simulink model "FullFMS_2026_02_25_V0_4_25_R2025b"  (R2025b)
settings: Solver=FixedStepAuto  StopTime=inf  FixedStep=0.01  MaxStep=0.01  RelTol=1e-2
PreLoadFcn:
  | load("BUS_CONFIG.mat")
libraries: opcualib x8
(part 2 of 4)

== matlab function FullFMS_2026_02_25_V0_4_25_R2025b/MATLAB Function6 ==
  data: F_92_Claw_2_Cart output boolean; F_92_Claw_2_Del output boolean; F_92_Claw_Down output boolean; F_92_Close_Claw output boolean; F_93_Led_Start output boolean; F_93_Led_Reset output boolean; F_93_Led_Extra1 output boolean; F_93_Led_Extra2 output boolean; F_93_Panel_O4 output boolean; F_93_Panel_O5 output boolean; F_93_Panel_O6 output boolean; F_93_Panel_O7 output boolean; u1 input boolean; A_94_Request output boolean; u2 input boolean; u3 input boolean; u4 input boolean; u5 input boolean; u6 input boolean; u7 input boolean; u8 input boolean; u9 input boolean; u10 input boolean; u11 input boolean; u12 input boolean; u13 input boolean; u14 input boolean; u15 input boolean; u16 input boolean; u17 input double; u18 input boolean; u19 input boolean; u20 input boolean; u21 input boolean; u22 input boolean; u23 input boolean; u24 input boolean; u25 input boolean; u26 input boolean; u27 input boolean; u28 input boolean; u29 input boolean; u30 input boolean; u31 input boolean; u32 input boolean; u33 input boolean; u34 input boolean; u35 input boolean; u36 input boolean; u37 input boolean; u38 input boolean; u39 input boolean; u40 input boolean; u41 input boolean; u42 input boolean; u43 input boolean; u44 input boolean; u45 input boolean; u46 input boolean; A_94_No_Cart output boolean; A_94_Cart_Full output boolean; A_94_CRoute_Out output boolean; A_93_ProcCartID output double; A_94_Cart_Stat output boolean; A_94_Cart_Next output boolean; A_94_Optic output boolean; A_94_Count output boolean; A_94_Pist_Bck output boolean; A_94_Release_FB output boolean; A_94_CRoute_In output boolean; C_95_Initialization output boolean; C_95_PD_Proc output boolean; C_95_PD_Cart output boolean; C_92_Profibus output boolean; C_95_Start output boolean; C_95_Cart2Del output boolean; C_95_Del2Cart output boolean; O_90_Part_Reserve output boolean; O_90_Claw_Del output boolean; O_90_Claw_Cart output boolean; O_90_Claw_Reserve output boolean; O_90_Claw_Low output boolean; O_90_Claw_High output boolean; O_90_Part_in_Claw output boolean; O_91_Start output boolean; O_91_Stop output boolean; O_91_Key_Pos output boolean; O_91_Reset output boolean; O_91_Panel_I4 output boolean; O_91_Panel_I5 output boolean; O_91_Panel_I6 output boolean; O_91_Panel_I7 output boolean
function [F_92_Claw_2_Cart,F_92_Claw_2_Del,F_92_Claw_Down,F_92_Close_Claw,F_93_Led_Start,F_93_Led_Reset,F_93_Led_Extra1,F_93_Led_Extra2,F_93_Panel_O4,F_93_Panel_O5,F_93_Panel_O6,F_93_Panel_O7, ...
    A_94_Request,A_94_No_Cart,A_94_Cart_Full,A_94_CRoute_Out,A_93_ProcCartID,A_94_Cart_Stat,A_94_Cart_Next,A_94_Optic,A_94_Count,A_94_Pist_Bck,A_94_Release_FB,A_94_CRoute_In, ...
    C_95_Initialization,C_95_PD_Proc,C_95_PD_Cart,C_92_Profibus,C_95_Start,C_95_Cart2Del,C_95_Del2Cart, ...
    O_90_Part_Reserve,O_90_Claw_Del,O_90_Claw_Cart,O_90_Claw_Reserve,O_90_Claw_Low,O_90_Claw_High,O_90_Part_in_Claw,O_91_Start,O_91_Stop,O_91_Key_Pos,O_91_Reset,O_91_Panel_I4,O_91_Panel_I5,O_91_Panel_I6,O_91_Panel_I7] = ...
    Handling2_90(u1, u2, u3, u4, u5, u6, u7, u8, u9, u10, u11, u12, u13, u14, u15, u16, u17, u18, u19, u20, u21, u22, u23, u24, u25, u26, u27, u28, u29, u30, u31, u32, u33, u34, u35, u36, u37, u38, u39, u40, u41, u42, u43, u44, u45, u46)

% Actuators (12 variables, starts at u1)
F_92_Claw_2_Cart = u1;
F_92_Claw_2_Del = u2;
F_92_Claw_Down = u3;
F_92_Close_Claw = u4;
F_93_Led_Start = u5;
F_93_Led_Reset = u6;
F_93_Led_Extra1 = u7;
F_93_Led_Extra2 = u8;
F_93_Panel_O4 = u9;
F_93_Panel_O5 = u10;
F_93_Panel_O6 = u11;
F_93_Panel_O7 = u12;

% AS-i (12 variables, starts at u13)
A_94_Request = u13;
A_94_No_Cart = u14;
A_94_Cart_Full = u15;
A_94_CRoute_Out = u16;
A_93_ProcCartID = u17;
A_94_Cart_Stat = u18;
A_94_Cart_Next = u19;
A_94_Optic = u20;
A_94_Count = u21;
A_94_Pist_Bck = u22;
A_94_Release_FB = u23;
A_94_CRoute_In = u24;

% Control (7 variables, starts at u25)
C_95_Initialization = u25;
C_95_PD_Proc = u26;
C_95_PD_Cart = u27;
C_92_Profibus = u28;
C_95_Start = u29;
C_95_Cart2Del = u30;
C_95_Del2Cart = u31;

% Sensors (15 variables, starts at u32)
O_90_Part_Reserve = u32;
O_90_Claw_Del = u33;
O_90_Claw_Cart = u34;
O_90_Claw_Reserve = u35;
O_90_Claw_Low = u36;
O_90_Claw_High = u37;
O_90_Part_in_Claw = u38;
O_91_Start = u39;
O_91_Stop = u40;
O_91_Key_Pos = u41;
O_91_Reset = u42;
O_91_Panel_I4 = u43;
O_91_Panel_I5 = u44;
O_91_Panel_I6 = u45;
O_91_Panel_I7 = u46;

end

== matlab function FullFMS_2026_02_25_V0_4_25_R2025b/MATLAB Function5 ==
  data: u1 input boolean; u2 input boolean; u3 input boolean; u4 input boolean; u5 input boolean; u6 input boolean; u7 input boolean; u8 input boolean; u9 input boolean; u10 input boolean; u11 input boolean; u12 input boolean; u13 input boolean; u14 input boolean; u15 input boolean; u16 input boolean; u17 input double; u18 input double; u19 input boolean; u20 input double; u21 input boolean; u22 input boolean; u23 input boolean; u24 input boolean; u25 input boolean; u26 input boolean; u27 input boolean; u28 input boolean; u29 input boolean; u30 input boolean; u31 input boolean; u32 input boolean; u33 input boolean; u34 input boolean; u35 input boolean; u36 input boolean; u37 input boolean; u38 input boolean; u39 input boolean; F_82_Pist_Adv output boolean; F_82_Suction_On output boolean; F_82_Suction_Off output boolean; F_82_Arm_2_Del output boolean; F_82_Arm_2_Mag output boolean; F_83_Led_Start output boolean; F_83_Led_Reset output boolean; F_83_Led_Extra1 output boolean; F_83_Led_Extra2 output boolean; F_83_Panel_O4 output boolean; F_83_Panel_O5 output boolean; F_83_Panel_O6 output boolean; F_83_Panel_O7 output boolean; C_85_Initialization output boolean; C_85_Part_Del output boolean; C_85_Part_Mag output boolean; C_86_Mag_Parts output double; C_87_RQ_MParts output double; C_82_Profibus output boolean; C_83_RQ_Parts output double; C_85_Start output boolean; C_85_Single output boolean; C_85_Continuous output boolean; C_85_Counted output boolean; O_80_Mag_Full output boolean; O_80_Pist_Bck output boolean; O_80_Pist_Fwd output boolean; O_80_Part_Stuck output boolean; O_80_Arm_Mag output boolean; O_80_Arm_Del output boolean; O_80_Mag_Empty output boolean; O_81_Start output boolean; O_81_Stop output boolean; O_81_Key_Pos output boolean; O_81_Reset output boolean; O_81_Panel_I4 output boolean; O_81_Panel_I5 output boolean; O_81_Panel_I6 output boolean; O_81_Panel_I7 output boolean
function [F_82_Pist_Adv, F_82_Suction_On,F_82_Suction_Off,F_82_Arm_2_Del,F_82_Arm_2_Mag,F_83_Led_Start , F_83_Led_Reset , F_83_Led_Extra1 , F_83_Led_Extra2 , F_83_Panel_O4 , F_83_Panel_O5 , F_83_Panel_O6 , F_83_Panel_O7, ...
    C_85_Initialization,C_85_Part_Del,C_85_Part_Mag,C_86_Mag_Parts,C_87_RQ_MParts,C_82_Profibus,C_83_RQ_Parts,C_85_Start,C_85_Single,C_85_Continuous,C_85_Counted, ...
    O_80_Mag_Full,O_80_Pist_Bck,O_80_Pist_Fwd,O_80_Part_Stuck,O_80_Arm_Mag,O_80_Arm_Del,O_80_Mag_Empty,O_81_Start,O_81_Stop,O_81_Key_Pos,O_81_Reset,O_81_Panel_I4,O_81_Panel_I5,O_81_Panel_I6,O_81_Panel_I7] = ...
    Distribution_80 (u1, u2, u3, u4, u5, u6, u7, u8, u9, u10, u11, u12, u13, u14, u15, u16, u17, u18, u19, u20, u21, u22, u23, u24, u25, u26, u27, u28, u29, u30, u31, u32, u33, u34, u35, u36, u37, u38, u39)

% Actuatorss (13 variables, starts at u1)
F_82_Pist_Adv = u1;
F_82_Suction_On = u2;
F_82_Suction_Off = u3;
F_82_Arm_2_Del = u4;
F_82_Arm_2_Mag = u5;
F_83_Led_Start = u6;
F_83_Led_Reset = u7;
F_83_Led_Extra1 = u8;
F_83_Led_Extra2 = u9;
F_83_Panel_O4 = u10;
F_83_Panel_O5 = u11;
F_83_Panel_O6 = u12;
F_83_Panel_O7 = u13;

% Control (11 varaibles, starts at u14)
C_85_Initialization = u14;
C_85_Part_Del = u15;
C_85_Part_Mag = u16;
C_86_Mag_Parts = u17;
C_87_RQ_MParts = u18;
C_82_Profibus = u19;
C_83_RQ_Parts = u20;
C_85_Start = u21;
C_85_Single = u22;
C_85_Continuous = u23;
C_85_Counted = u24;

% Sensors (15 variables, starts at u25)
O_80_Mag_Full = u25;
O_80_Pist_Bck = u26;
O_80_Pist_Fwd = u27;
O_80_Part_Stuck = u28;
O_80_Arm_Mag = u29;
O_80_Arm_Del = u30;
O_80_Mag_Empty = u31;
O_81_Start = u32;
O_81_Stop = u33;
O_81_Key_Pos = u34;
O_81_Reset = u35;
O_81_Panel_I4 = u36;
O_81_Panel_I5 = u37;
O_81_Panel_I6 = u38;
O_81_Panel_I7 = u39;

end

== matlab function FullFMS_2026_02_25_V0_4_25_R2025b/MATLAB Function4 ==
  data: u1 input boolean; u2 input boolean; u3 input boolean; u4 input boolean; u5 input boolean; u6 input boolean; u7 input boolean; u8 input boolean; u9 input boolean; u10 input boolean; u11 input boolean; u12 input boolean; u13 input boolean; u14 input boolean; u15 input boolean; u16 input boolean; u17 input boolean; u18 input double; u19 input boolean; u20 input boolean; u21 input boolean; u22 input boolean; u23 input boolean; u24 input boolean; u25 input boolean; u26 input boolean; u27 input boolean; u28 input boolean; u29 input boolean; u30 input boolean; u31 input boolean; u32 input boolean; u33 input boolean; u34 input boolean; u35 input boolean; u36 input boolean; u37 input boolean; u38 input boolean; u39 input boolean; u40 input boolean; u41 input boolean; u42 input boolean; u43 input boolean; u44 input boolean; u45 input boolean; u46 input boolean; u47 input boolean; u48 input boolean; u49 input boolean; u50 input boolean; u51 input boolean; u52 input boolean; u53 input boolean; F_72_Elev_Down output boolean; F_72_Elev_Up output boolean; F_72_Eject_Part output boolean; F_72_Air_On output boolean; F_73_Led_Start output boolean; F_73_Led_Reset output boolean; F_73_Led_Extra1 output boolean; F_73_Led_Extra2 output boolean; F_73_Panel_O4 output boolean; F_73_Panel_O5 output boolean; F_73_Panel_O6 output boolean; F_73_Panel_O7 output boolean; A_74_Request output boolean; A_74_No_Cart output boolean; A_74_Cart_Full output boolean; A_74_CRoute_Out output boolean; A_74_CRoute_In80 output boolean; A_73_TestCartID output double; A_74_Cart_Stat output boolean; A_74_Cart_Next output boolean; A_74_Optic output boolean; A_74_Count output boolean; A_74_Pist_Bck output boolean; A_74_Release_FB output boolean; A_74_CRoute_In output boolean; C_75_Initialization output boolean; C_75_ID_Delivery1 output boolean; C_75_ID_Delivery2 output boolean; C_75_Part_Del output boolean; C_75_RQ_Part_Del output boolean; C_75_RQ_Wrong output boolean; C_75_Identified80 output boolean; C_75_Requested80 output boolean; C_72_Profibus output boolean; C_75_RQ_Delivery1 output boolean; C_75_RQ_Delivery2 output boolean; C_75_Identified output boolean; C_75_Requested output boolean; O_70_SInductive output boolean; O_70_SPart output boolean; O_70_SStation output boolean; O_70_SPart_Height output boolean; O_70_Elev_High output boolean; O_70_Elev_Low output boolean; O_70_Pist_Bck output boolean; O_71_Start output boolean; O_71_Stop output boolean; O_71_Key_Pos output boolean; O_71_Reset output boolean; O_71_Panel_I4 output boolean; O_71_Panel_I5 output boolean; O_71_Panel_I6 output boolean; O_71_Panel_I7 output boolean
function [F_72_Elev_Down,F_72_Elev_Up,F_72_Eject_Part,F_72_Air_On,F_73_Led_Start,F_73_Led_Reset,F_73_Led_Extra1,F_73_Led_Extra2,F_73_Panel_O4,F_73_Panel_O5,F_73_Panel_O6,F_73_Panel_O7, ...	
    A_74_Request,A_74_No_Cart,A_74_Cart_Full,A_74_CRoute_Out,A_74_CRoute_In80,A_73_TestCartID,A_74_Cart_Stat,A_74_Cart_Next,A_74_Optic,A_74_Count,A_74_Pist_Bck,A_74_Release_FB,A_74_CRoute_In, ...
    C_75_Initialization,C_75_ID_Delivery1,C_75_ID_Delivery2,C_75_Part_Del,C_75_RQ_Part_Del,C_75_RQ_Wrong,C_75_Identified80,C_75_Requested80,C_72_Profibus,C_75_RQ_Delivery1,C_75_RQ_Delivery2,C_75_Identified , C_75_Requested, ...
    O_70_SInductive,O_70_SPart,O_70_SStation,O_70_SPart_Height,O_70_Elev_High,O_70_Elev_Low,O_70_Pist_Bck,O_71_Start,O_71_Stop,O_71_Key_Pos,O_71_Reset,O_71_Panel_I4,O_71_Panel_I5,O_71_Panel_I6,O_71_Panel_I7] = ...
    Testing_70(u1, u2, u3, u4, u5, u6, u7, u8, u9, u10, u11, u12, u13, u14, u15, u16, u17, u18, u19, u20, u21, u22, u23, u24, u25, u26, u27, u28, u29, u30, u31, u32, u33, u34, u35, u36, u37, u38, u39, u40, u41, u42, u43, u44, u45, u46, u47, u48, u49, u50, u51, u52, u53)

% Actuators (12 variables, starts at u1)
F_72_Elev_Down = u1;
F_72_Elev_Up = u2;
F_72_Eject_Part = u3;
F_72_Air_On = u4;
F_73_Led_Start = u5;
F_73_Led_Reset = u6;
F_73_Led_Extra1 = u7;
F_73_Led_Extra2 = u8;
F_73_Panel_O4 = u9;
F_73_Panel_O5 = u10;
F_73_Panel_O6 = u11;
F_73_Panel_O7 = u12;

% AS-i (13 varaibles, starts at u13)
A_74_Request = u13;
A_74_No_Cart = u14;
A_74_Cart_Full = u15;
A_74_CRoute_Out = u16;
A_74_CRoute_In80 = u17;
A_73_TestCartID = u18;
A_74_Cart_Stat = u19;
A_74_Cart_Next = u20;
A_74_Optic = u21;
A_74_Count = u22;
A_74_Pist_Bck = u23;
A_74_Release_FB = u24;
A_74_CRoute_In = u25;

% Control (13 variables, starts at u26)
C_75_Initialization = u26;
C_75_ID_Delivery1 = u27;
C_75_ID_Delivery2 = u28;
C_75_Part_Del = u29;
C_75_RQ_Part_Del = u30;
C_75_RQ_Wrong = u31;
C_75_Identified80 = u32;
C_75_Requested80 = u33;
C_72_Profibus = u34;
C_75_RQ_Delivery1 = u35;
C_75_RQ_Delivery2 = u36;
C_75_Identified = u37;
C_75_Requested = u38;

% Sensors (15 variables, starts at u39)
O_70_SInductive = u39;
O_70_SPart = u40;
O_70_SStation = u41;
O_70_SPart_Height = u42;
O_70_Elev_High = u43;
O_70_Elev_Low = u44;
O_70_Pist_Bck = u45;
O_71_Start = u46;
O_71_Stop = u47;
O_71_Key_Pos = u48;
O_71_Reset = u49;
O_71_Panel_I4 = u50;
O_71_Panel_I5 = u51;
O_71_Panel_I6 = u52;
O_71_Panel_I7 = u53;

end

== matlab function FullFMS_2026_02_25_V0_4_25_R2025b/MATLAB Function7 ==
  data: F_102_Drill_On output boolean; F_102_RT_On output boolean; F_102_Drill_Down output boolean; F_102_Drill_Up output boolean; F_102_Drill_Pin output boolean; F_102_Test_Pin output boolean; F_103_Led_Start output boolean; F_103_Led_Reset output boolean; F_103_Led_Extra1 output boolean; F_103_Led_Extra2 output boolean; F_103_Panel_O4 output boolean; F_103_Panel_O5 output boolean; F_103_Panel_O6 output boolean; F_103_Panel_O7 output boolean; u1 input boolean; C_105_Initialization output boolean; u2 input boolean; u3 input boolean; u4 input boolean; u5 input boolean; u6 input boolean; u7 input boolean; u8 input boolean; u9 input boolean; u10 input boolean; u11 input boolean; u12 input boolean; u13 input boolean; u14 input boolean; u15 input boolean; u16 input boolean; u17 input boolean; u18 input boolean; u19 input double; u20 input boolean; u21 input double; u22 input boolean; u23 input boolean; u24 input boolean; u25 input boolean; u26 input boolean; u27 input boolean; u28 input boolean; u29 input boolean; u30 input boolean; u31 input boolean; u32 input boolean; u33 input boolean; u34 input boolean; u35 input boolean; u36 input boolean; u37 input boolean; u38 input boolean; u39 input boolean; C_105_Part_ready output boolean; C_105_Test_Ok output boolean; C_105_Test_Fail output boolean; C_106_RT_Counter output double; C_102_Profibus output boolean; C_103_RQ_Turns output double; C_105_Start output boolean; C_105_Test output boolean; C_105_TestDrill output boolean; C_105_Rotation output boolean; O_100_PInit_Pos output boolean; O_100_PDrill_Pos output boolean; O_100_PTest_Pos output boolean; O_100_SDrill_High output boolean; O_100_SDrill_Low output boolean; O_100_RT_Sensor output boolean; O_100_PTest_Ok output boolean; O_101_Start output boolean; O_101_Stop output boolean; O_101_Key_Pos output boolean; O_101_Reset output boolean; O_101_Panel_I4 output boolean; O_101_Panel_I5 output boolean; O_101_Panel_I6 output boolean; O_101_Panel_I7 output boolean; u40 input boolean
function [F_102_Drill_On,F_102_RT_On,F_102_Drill_Down,F_102_Drill_Up,F_102_Drill_Pin,F_102_Test_Pin,F_103_Led_Start,F_103_Led_Reset,F_103_Led_Extra1,F_103_Led_Extra2,F_103_Panel_O4,F_103_Panel_O5,F_103_Panel_O6,F_103_Panel_O7, ...
    C_105_Initialization,C_105_Part_ready,C_105_Test_Ok,C_105_Test_Fail,C_106_RT_Counter,C_102_Profibus,C_103_RQ_Turns,C_105_Start,C_105_Test,C_105_TestDrill,C_105_Rotation, ...
    O_100_PInit_Pos,O_100_PDrill_Pos,O_100_PTest_Pos,O_100_SDrill_High,O_100_SDrill_Low,O_100_RT_Sensor,O_100_PTest_Ok,O_101_Start,O_101_Stop,O_101_Key_Pos,O_101_Reset,O_101_Panel_I4,O_101_Panel_I5,O_101_Panel_I6,O_101_Panel_I7] = ...
    Processing_100(u1, u2, u3, u4, u5, u6, u7, u8, u9, u10, u11, u12, u13, u14, u15, u16, u17, u18, u19, u20, u21, u22, u23, u24, u25, u26, u27, u28, u29, u30, u31, u32, u33, u34, u35, u36, u37, u38, u39, u40)

% Actuators (14 variables, starts at u1)
F_102_Drill_On = u1;
F_102_RT_On = u2;
F_102_Drill_Down = u3;
F_102_Drill_Up = u4;
F_102_Drill_Pin = u5;
F_102_Test_Pin = u6;
F_103_Led_Start = u7;
F_103_Led_Reset = u8;
F_103_Led_Extra1 = u9;
F_103_Led_Extra2 = u10;
F_103_Panel_O4 = u11;
F_103_Panel_O5 = u12;
F_103_Panel_O6 = u13;
F_103_Panel_O7 = u14;

% Control (11 variables, starting at u15)
C_105_Initialization = u15;
C_105_Part_ready = u16;
C_105_Test_Ok = u17;
C_105_Test_Fail = u18;
C_106_RT_Counter = u19;
C_102_Profibus = u20;
C_103_RQ_Turns = u21;
C_105_Start = u22;
C_105_Test = u23;
C_105_TestDrill = u24;
C_105_Rotation = u25;

% Sensors (15 variables, starts at u26)
O_100_PInit_Pos = u26;
O_100_PDrill_Pos = u27;
O_100_PTest_Pos = u28;
O_100_SDrill_High = u29;
O_100_SDrill_Low = u30;
O_100_RT_Sensor = u31;
O_100_PTest_Ok = u32;
O_101_Start = u33;
O_101_Stop = u34;
O_101_Key_Pos = u35;
O_101_Reset = u36;
O_101_Panel_I4 = u37;
O_101_Panel_I5 = u38;
O_101_Panel_I6 = u39;
O_101_Panel_I7 = u40;

end

== matlab function FullFMS_2026_02_25_V0_4_25_R2025b/MATLAB Function8 ==
  data: u1 input boolean; u2 input boolean; u3 input boolean; u4 input boolean; u5 input boolean; u6 input boolean; u7 input boolean; u8 input boolean; u9 input boolean; u10 input boolean; u11 input boolean; u12 input boolean; u13 input double; u14 input boolean; u15 input boolean; u16 input boolean; u17 input boolean; u18 input boolean; u19 input boolean; u20 input boolean; u21 input boolean; u22 input boolean; u23 input boolean; u24 input boolean; u25 input boolean; u26 input boolean; u27 input boolean; u28 input boolean; u29 input boolean; u30 input boolean; u31 input boolean; u32 input boolean; u33 input boolean; F_43_Led_Start output boolean; F_43_Led_Reset output boolean; F_43_Led_Extra1 output boolean; F_43_Led_Extra2 output boolean; F_43_Panel_O4 output boolean; F_43_Panel_O5 output boolean; F_43_Panel_O6 output boolean; F_43_Panel_O7 output boolean; A_44_Request output boolean; A_44_No_Cart output boolean; A_44_Cart_Full output boolean; A_44_CRoute_Out output boolean; A_43_StorCartID output double; A_44_Cart_Stat output boolean; A_44_Cart_Next output boolean; A_44_Optic output boolean; A_44_Count output boolean; A_44_Pist_Bck output boolean; A_44_Release_FB output boolean; A_44_CRoute_In output boolean; C_45_Initialization output boolean; C_42_Profibus output boolean; C_45_Start output boolean; C_45_StorePart output boolean; C_45_RetrievePart output boolean; O_41_Start output boolean; O_41_Stop output boolean; O_41_Key_Pos output boolean; O_41_Reset output boolean; O_41_Panel_I4 output boolean; O_41_Panel_I5 output boolean; O_41_Panel_I6 output boolean; O_41_Panel_I7 output boolean
function [F_43_Led_Start,F_43_Led_Reset,F_43_Led_Extra1,F_43_Led_Extra2,F_43_Panel_O4,F_43_Panel_O5,F_43_Panel_O6,F_43_Panel_O7,...
 A_44_Request,A_44_No_Cart,A_44_Cart_Full,A_44_CRoute_Out,A_43_StorCartID,A_44_Cart_Stat,A_44_Cart_Next,A_44_Optic,A_44_Count,A_44_Pist_Bck,A_44_Release_FB,A_44_CRoute_In,...
 C_45_Initialization,C_42_Profibus,C_45_Start,C_45_StorePart,C_45_RetrievePart,...
    O_41_Start,O_41_Stop,O_41_Key_Pos,O_41_Reset,O_41_Panel_I4,O_41_Panel_I5,O_41_Panel_I6,O_41_Panel_I7] = ...
    Storage_40 (u1, u2, u3, u4, u5, u6, u7, u8, u9, u10, u11, u12, u13, u14, u15, u16, u17, u18, u19, u20, u21, u22, u23, u24, u25, u26, u27, u28, u29, u30, u31, u32, u33)

% Actuators (8 variables: starts at u1)
F_43_Led_Start = u1;
F_43_Led_Reset = u2;
F_43_Led_Extra1 = u3; 
F_43_Led_Extra2 = u4;
F_43_Panel_O4 = u5;
F_43_Panel_O5 = u6;
F_43_Panel_O6 = u7;
F_43_Panel_O7 = u8;

% AS-i (12 variables: starts at u9)
A_44_Request = u9;
A_44_No_Cart = u10;
A_44_Cart_Full = u11;
A_44_CRoute_Out = u12;
A_43_StorCartID = u13;
A_44_Cart_Stat = u14;
A_44_Cart_Next = u15;
A_44_Optic = u16;
A_44_Count = u17;
A_44_Pist_Bck = u18;
A_44_Release_FB = u19;
A_44_CRoute_In = u20;

% Control (5 variables: starts at u21)
C_45_Initialization = u21;
C_42_Profibus = u22;
C_45_Start = u23;
C_45_StorePart = u24;
C_45_RetrievePart = u25;

% Sensors (8 variables: starts at u26)
O_41_Start = u26;
O_41_Stop = u27;
O_41_Key_Pos = u28;
O_41_Reset = u29;
O_41_Panel_I4 = u30;
O_41_Panel_I5 = u31;
O_41_Panel_I6 = u32;
O_41_Panel_I7 = u33;

end
